simulink model "dummy"  (Simulink 6.5)
settings: Solver=FixedStepDiscrete  StartTime=0.0  StopTime=inf  FixedStep=0.001  RelTol=1e-3
PreLoadFcn:
  | RTWConfigurationCB('preloadfcn', bdroot);
InitFcn:
  | % END RTW CONFIGURATION CODE %
libraries: dsPICdrivers x8
CloseFcn:
  | rtwprivate ssgencode ModelCloseRequest LVTest2
settings Model: Creator=admin-wmg139  LastModifiedBy=Bernard Leak  BufferReuse=off  ProdHWDeviceType=16-bit Generic
settings DataIOCC: SaveTime=off  SignalLoggingName=sigsOut
settings OptimizationCC: BlockReduction=off  OptimizeBlockIOStorage=off  BufferReuse=off  ExpressionFolding=off  LocalBlockOutputs=off  NoFixptDivByZeroProtection=on  EfficientFloat2IntCast=on  OptimizeModelRefInitCode=on  LifeSpan=1
settings DebuggingCC: SolverPrmCheckMsg=none  MultiTaskDSMMsg=warning  MultiTaskCondExecSysMsg=none  StrictBusMsg=None
settings HardwareCC: ProdBitPerInt=16  ProdEndianess=LittleEndian  ProdWordSize=16  ProdHWDeviceType=16-bit Generic  TargetHWDeviceType=32-bit Generic
settings RTWCC: SystemTargetFile=dspic.tlc  TemplateMakefile=dspic_pic30_gcc.tmf  PostCodeGenCommand=dsPIC_Compile()  Description=Embedded Target for Microchip dsPIC (real-time)  RetainRTWFile=on  ProcessScript=dspic_make_rtw_hook  IncludeERTFirstTime=on
settings CodeAppCC: IgnoreCustomStorageClasses=off
settings STFCustomTargetCC: TargetFcnLib=ansi_tfl_tmw.mat  GenFloatMathFcnCalls=ANSI_C  ModelReferenceCompliant=off  IncludeMdlTerminateFcn=off  CombineOutputUpdateFcns=on  SuppressErrorStatus=on  ERTCustomFileBanners=on  SupportContinuousTime=off  SupportNonInlinedSFcns=off  SystemTargetFile=dspic.tlc
settings ERTTargetCC: TargetFcnLib=ansi_tfl_tmw.mat  GenFloatMathFcnCalls=ANSI_C  ModelReferenceCompliant=off  IncludeMdlTerminateFcn=off  SuppressErrorStatus=on  InlinedParameterPlacement=NonHierarchical  ERTSrcFileBannerTemplate=dsPIC_code_template.cgt  ERTHdrFileBannerTemplate=dsPIC_code_template.cgt  ERTDataSrcFileTemplate=dsPIC_code_template.cgt  ERTDataHdrFileTemplate=dsPIC_code_template.cgt  ERTCustomFileTemplate=dsPIC_main.tlc
settings CustomProperty: DataType=string  Value=C:\MATLAB6b\rtw\bin\win32\gmake

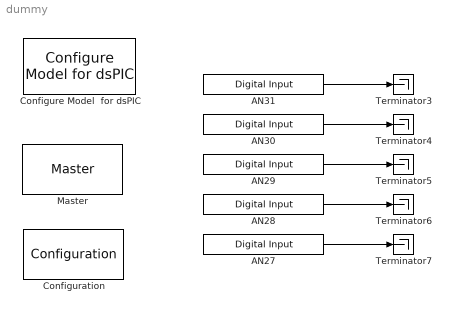
== system dummy ==
  AN27 : dsPICdrivers/Digital I//O/Digital Input  Tag=dsPIC_Digital_Input  PORT=E  Pin=[3]  SampleTime=inf  OrderingInOutPopup=None
  AN28 : dsPICdrivers/Digital I//O/Digital Input  Tag=dsPIC_Digital_Input  PORT=E  Pin=[4]  SampleTime=inf  OrderingInOutPopup=None
  AN29 : dsPICdrivers/Digital I//O/Digital Input  Tag=dsPIC_Digital_Input  PORT=E  Pin=[5]  SampleTime=inf  OrderingInOutPopup=None
  AN30 : dsPICdrivers/Digital I//O/Digital Input  Tag=dsPIC_Digital_Input  PORT=E  Pin=[6]  SampleTime=inf  OrderingInOutPopup=None
  AN31 : dsPICdrivers/Digital I//O/Digital Input  Tag=dsPIC_Digital_Input  PORT=E  Pin=[7]  SampleTime=inf  OrderingInOutPopup=None
  Configuration : dsPICdrivers/Configuration  SystemSampleTime=-1  double64=on
  Configure Model  for dsPIC : dsPICdrivers/Simulink Configuration/Configure Model  for dsPIC
  Master : dsPICdrivers/Master  Tag=dsPIC_MASTER  Priority=1  TimeStepType=Timer1  picType=33fJ256GP710  fcy=5000000  Quartz_33f=1e7  PLLActive_33f=off  fcyDesired_33f=1e7  tmr1="[1  39999  0]"  tmr1Info="Time Step : 0.001  ;   Error : 0%  PR1=39999"  tmr2345="[0  0  0  0  0  0  0  0]"  tmr2345cfg=[-1 -1 -1 -1 -1 -1 -1 -1]  IOautoConf=on  typePort="[ 0  0  0  0  0  0  0  0  0  0  0  0  0  0  0  0  0  0  0  0  0  0  0  0  0  0  0  0  0  0  0  0  0  0  0  0  0  0  0  0  0  0  0  0  0  0  0  0  0  0  0  0  0  0  0  0  0  0  0  0  0  0  0  0  0  0  0  9  9  9  9  9  0  0  0  0  0  0  0  0  0  0  0  0  0  0  0  0  0  0  0  0  0  0  0  0  0  0  0  0  0  0  0  0  0  0  0  0  0  0  0  0 ]"  TRIS="[ 65535  65535  65535  65535  65535  65535  65535 ]"  ADPCFG=4160749568  MasterBusyPort=None  MasterOverloadPort=None  FOSC=Quartz (XT - HS)  ClockSwitchMonitor=Clock switching and monitor enabled  TempProtection_33f=TEMP_ON  FPBOR=<empty>  PWRT=64ms  MCLR=<empty>  PowerSave=off  OverrideFcy=on  NewFcy=4e7  PR2345="[65535  65535  65535  65535  65535  65535  65535  65535]"
  Terminator{3..7} (5 alike) : Terminator
  wires:
  AN31/1 -> Terminator3/1
  AN30/1 -> Terminator4/1
  AN29/1 -> Terminator5/1
  AN28/1 -> Terminator6/1
  AN27/1 -> Terminator7/1
